simulink model "Inversor_Real"  (R2026b)
settings: Solver=VariableStepAuto
values from neighbouring files (symbols this model uses):
  sat_V = sqrt(2/3)*V_slMAX    [coeficientes.m]
libraries: eeGeneralControl x3
settings Model: Creator=fedeb  LastModifiedBy=fedeb

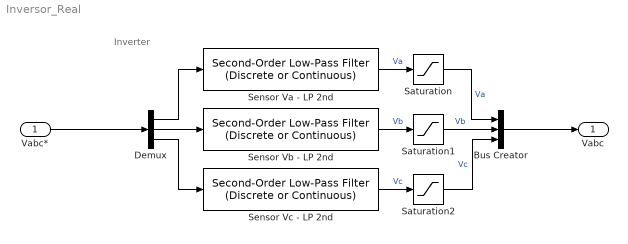
== system Inversor_Real ==
  note: Inverter
  Vabc* : Inport
  Bus Creator : BusCreator  Inputs=3
  Demux : Demux  Outputs=3
  Saturation : Saturate  UpperLimit=sat_V  LowerLimit=-sat_V
  Saturation1 : Saturate  UpperLimit=sat_V  LowerLimit=-sat_V
  Saturation2 : Saturate  UpperLimit=sat_V  LowerLimit=-sat_V
  Sensor Va - LP 2nd : eeGeneralControl/Second-Order Low-Pass Filter (Discrete or Continuous)  A1=A1_V  A2=A2_V  init_option=Inherited from block input  x0=0  Ts=0
      settings: LibrarySourceBlock=|
      | ee_sl_lib/General Control/Second-Order
      | Low-Pass Filter
      | (Discrete or Continuous)
  Sensor Vb - LP 2nd : eeGeneralControl/Second-Order Low-Pass Filter (Discrete or Continuous)  A1=A1_V  A2=A2_V  init_option=Inherited from block input  x0=0  Ts=0
      settings: LibrarySourceBlock=|
      | ee_sl_lib/General Control/Second-Order
      | Low-Pass Filter
      | (Discrete or Continuous)
  Sensor Vc - LP 2nd : eeGeneralControl/Second-Order Low-Pass Filter (Discrete or Continuous)  A1=A1_V  A2=A2_V  init_option=Inherited from block input  x0=0  Ts=0
      settings: LibrarySourceBlock=|
      | ee_sl_lib/General Control/Second-Order
      | Low-Pass Filter
      | (Discrete or Continuous)
  Vabc : Outport
  wires:
  Vabc*/1 -> Demux/1
  Demux/2 -> Sensor Vb - LP 2nd/1
  Demux/1 -> Sensor Va - LP 2nd/1
  Demux/3 -> Sensor Vc - LP 2nd/1
  Bus Creator/1 -> Vabc/1
  Sensor Va - LP 2nd/1 -> Saturation/1  "Va"
  Sensor Vb - LP 2nd/1 -> Saturation1/1  "Vb"
  Sensor Vc - LP 2nd/1 -> Saturation2/1  "Vc"
  Saturation2/1 -> Bus Creator/3  "Vc"
  Saturation1/1 -> Bus Creator/2  "Vb"
  Saturation/1 -> Bus Creator/1  "Va"
